simulink model "control_logic"  (R2025b)
settings: Solver=FixedStepDiscrete  StartTime=0.0  StopTime=30  FixedStep=0.1  RelTol=1e-3  EnableMultiTasking=on
settings Model: Creator=mayak  LastModifiedBy=fatim
settings SolverCC: AlgebraicLoopSolver=TrustRegion  AutoInsertRateTranBlk=on
settings DataIOCC: LimitDataPoints=on
settings OptimizationCC: LifeSpan=inf
settings DebuggingCC: UnconnectedInputMsg=warning  UnconnectedOutputMsg=warning  UnconnectedLineMsg=warning  AllowSymbolicDim=off  SFUnexpectedBacktrackingDiag=warning  SFNoUnconditionalDefaultTransitionDiag=warning  SFExecutionAtInitializationDiag=none  ArithmeticOperatorsInVariantConditions=warning
settings ModelReferenceCC: EnableRefExpFcnMdlSchedulingChecks=on
settings SFSimCC: SimUseLocalCustomCode=off  CustomCodeUndefinedFunction=UseInterfaceOnly
settings RTWCC: RTWUseLocalCustomCode=off  GPUComputeCapability=3.5  DLArmComputeVersion=19.05
settings CodeAppCC: StateflowObjectComments=on
settings GRTTargetCC: TargetLangStandard=C89/C90 (ANSI)
settings ConfigComp: CovMetricSettings=dw  CovSaveCumulativeToWorkspaceVar=on  CovSaveSingleToWorkspaceVar=on  CovExternalEMLEnable=off  CovSFcnEnable=off

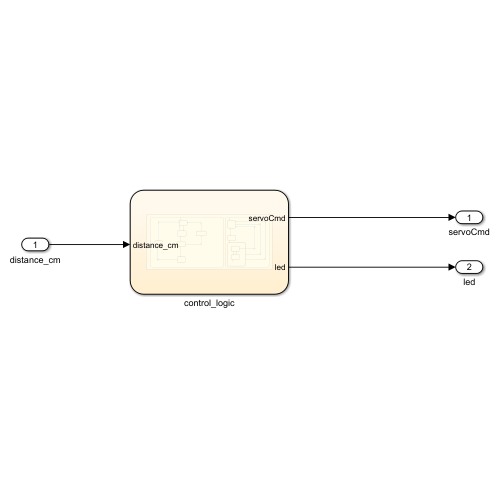
[thumbnail: Simulink's stored preview of the top-level diagram]
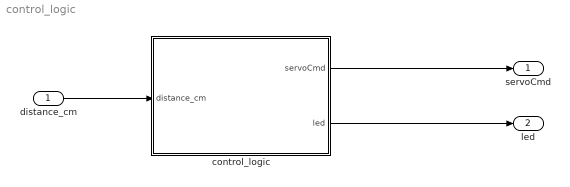
== system control_logic ==
  distance_cm : Inport
  control_logic : Stateflow chart  TreatAsAtomicUnit=on
  servoCmd : Outport
  led : Outport  Port=2
  wires:
  control_logic/1(servoCmd) -> servoCmd/1
  control_logic/2(led) -> led/1
  distance_cm/1 -> control_logic/1(distance_cm)

== stateflow chart control_logic/control_logic ==
  state control_logic
    state LID [parallel]
      settings: executionOrder=1
      state CLOSED
        entry:
        servoCmd=0;
      state DETECTION
        entry:
        servoCmd = 0;
        led = 0;
      state TIMEOUT
        entry:
        servoCmd=0;
      state WAIT
        entry:
        servoCmd=0;
        blink_cmd = 2;
      state HALF_OPEN
        entry:
        servoCmd=90;
        blink_cmd = 1;
      state OPEN
        entry:
        servoCmd=180;
        blink_cmd = 1;
      (default) -> CLOSED
      (junction 20) -> CLOSED
      (junction 64) -> CLOSED
      WAIT -> (junction 20) : after(30, sec){blink_cmd = 0; cnt = 0;}
      TIMEOUT -> (junction 64) : [distance_cm > 2.5]{blink_cmd = 0; cnt = 0;}
      DETECTION -> CLOSED [order 2] : [distance_cm <= 0.5 || distance_cm > 2.5]
      CLOSED -> DETECTION : [distance_cm > 0.5 && distance_cm <= 2.5]
      (junction 60) -> TIMEOUT : [duration(distance_cm > 1 && distance_cm <= 2.5, sec) >=10]{blink_cmd=999;}
      DETECTION -> HALF_OPEN [order 1] : [ duration(distance_cm > 0.5 && distance_cm <= 2.5, sec) >= 5 ]
      HALF_OPEN -> (junction 60) [order 2]
      (junction 19) -> WAIT : after(10,sec)
      HALF_OPEN -> OPEN [order 1] : [distance_cm <= 1 && temporalCount(sec) <= 10]
      OPEN -> (junction 19)
    state LED [parallel]
      settings: executionOrder=2
      state OFF
        entry:
        led=0
      state ON
        entry:
        led=1;
      state BLINKER
        state BLINK_OFF
          entry:
          led=0;
          cnt = cnt + 1;
        state BLINK_ON
          entry:
          led=1;
        BLINK_OFF -> BLINK_ON [order 1] : after(1, sec)
        BLINK_ON -> BLINK_OFF : after(1, sec)
        (default) -> BLINK_ON
      (default) -> OFF
      (junction 68) -> OFF
      (junction 67) -> (junction 68)
      OFF -> (junction 39) [order 1]
      (junction 39) -> (junction 40) : [blink_cmd > 0]
      (junction 56) -> OFF
      (junction 47) -> (junction 56)
      OFF -> ON [order 2] : [distance_cm<=0.5]
      ON -> BLINKER : [blink_cmd > 0]
      BLINK_OFF -> (junction 47) [order 2] : [cnt >= blink_cmd] {cnt = 0; blink_cmd = 0;}
      (junction 40) -> BLINKER
      BLINKER -> (junction 67) : [distance_cm > 2.5  && blink_cmd == 0]
  data: blink_cmd local =0; distance_cm input; servoCmd output; led output; cnt local =0
